simulink model "DiSiUp_1lab_3_2"  (R2025b)
settings: Solver=VariableStepAuto  StartTime=0.0  StopTime=100  RelTol=1e-8
values from neighbouring files (symbols this model uses):
  B_dist = [ ... (first row only)    [DiSiUp_lab1_3_2_mat.m]
  D_dist = 0    [DiSiUp_lab1_3_2_mat.m]
  Gamma_dist = [ ... (first row only)    [DiSiUp_lab1_3_2_mat.m]
  H_dist = [1, 0, 0, 0]    [DiSiUp_lab1_3_2_mat.m]
  T_dist = 0.25    [DiSiUp_lab1_3_2_mat.m]
  xi0_dist = [ ... (first row only)    [DiSiUp_lab1_3_2_mat.m]
settings Model: Creator=waltanmari  LastModifiedBy=waltanmari

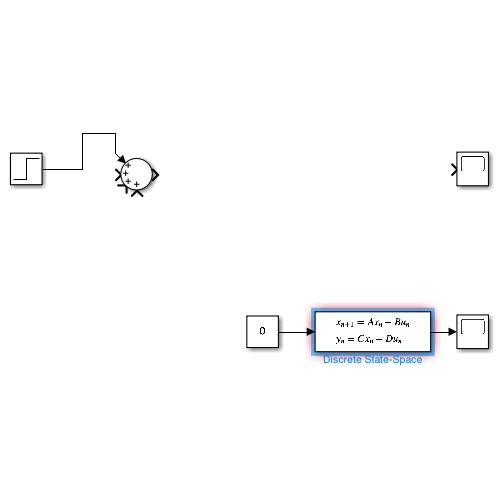
[thumbnail: Simulink's stored preview of the top-level diagram]
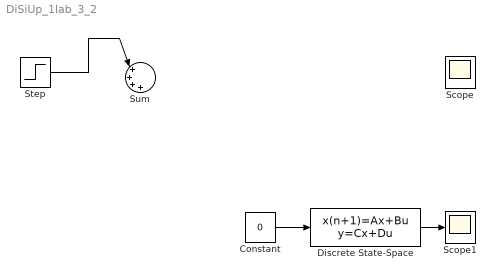
== system DiSiUp_1lab_3_2 ==
  Constant : Constant  Value=0
  Discrete State-Space : DiscreteStateSpace  A=Gamma_dist  B=B_dist  C=H_dist  D=D_dist  InitialCondition=xi0_dist  SampleTime=T_dist
  Scope : Scope
      settings: ActiveDisplayYMinimum=-1  ActiveDisplayYMaximum=1
  Scope1 : Scope
      settings: ActiveDisplayYMinimum=-1.5614219549727133  ActiveDisplayYMaximum=1.5385501108070716
  Step : Step  Time=0  After=0  SampleTime=0
  Sum : Sum  Inputs=|++++
  wires:
  Step/1 -> Sum/1
  Constant/1 -> Discrete State-Space/1
  Discrete State-Space/1 -> Scope1/1
